simulink library "Surface_Profile_Axle2_KnC"  (R2025a)
settings: Solver=VariableStepAuto  StartTime=0.0  StopTime=10.0  RelTol=1e-3
undefined symbols (not defined in the file): Maneuver
libraries: simulink x2
Description:
  | Simscape Vehicle Templates Library
  | 
  | Copyright 2018-2026 The MathWorks, Inc.
settings Model: Creator=smiller  LastModifiedBy=smiller
settings OptimizationCC: ReuseModelBlockBuffer=off
settings ModelReferenceCC: EnableRefExpFcnMdlSchedulingChecks=on
settings RTWCC: GPUComputeCapability=3.5

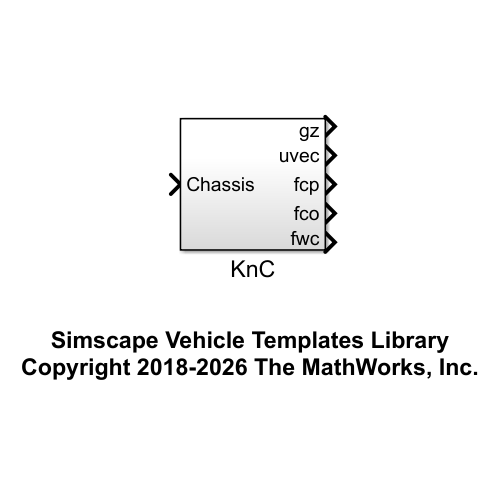
[thumbnail: Simulink's stored preview of the top-level diagram]
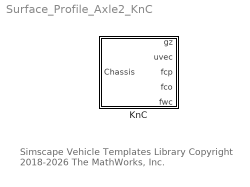
== system Surface_Profile_Axle2_KnC ==
  note: Simscape Vehicle Templates Library
      | Copyright 2018-2026 The MathWorks, Inc.
  KnC : Subsystem  VariantControl=KnC

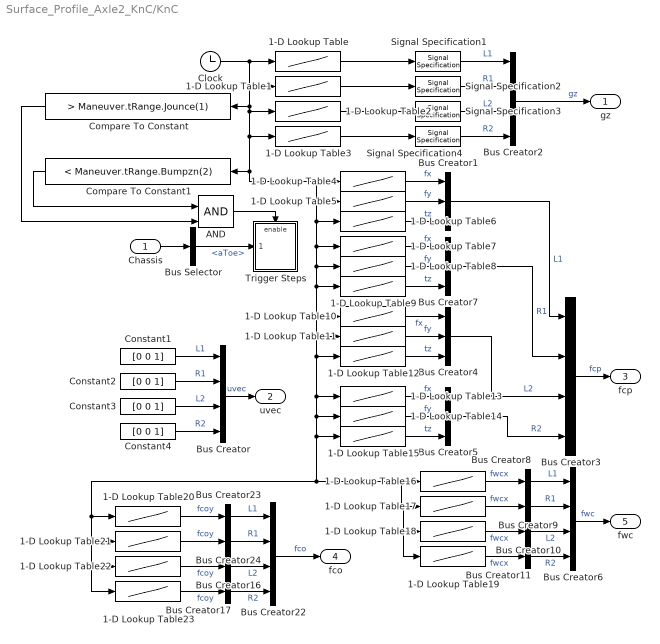
== system Surface_Profile_Axle2_KnC/KnC ==
  Chassis : Inport
  1-D Lookup Table : Lookup_n-D  NumberOfTableDimensions=1  BreakpointsForDimension1=Maneuver.PostL1.t.Value  Table=Maneuver.PostL1.z.Value  InternalRulePriority=Speed  RndMeth=Simplest
  1-D Lookup Table1 : Lookup_n-D  NumberOfTableDimensions=1  BreakpointsForDimension1=Maneuver.PostR1.t.Value  Table=Maneuver.PostR1.z.Value  InternalRulePriority=Speed  RndMeth=Simplest
  1-D Lookup Table10 : Lookup_n-D  NumberOfTableDimensions=1  BreakpointsForDimension1=Maneuver.PostL2.t.Value  Table=Maneuver.PostL2.fx.Value  InternalRulePriority=Speed  RndMeth=Simplest
  1-D Lookup Table11 : Lookup_n-D  NumberOfTableDimensions=1  BreakpointsForDimension1=Maneuver.PostL2.t.Value  Table=Maneuver.PostL2.fy.Value  InternalRulePriority=Speed  RndMeth=Simplest
  1-D Lookup Table12 : Lookup_n-D  NumberOfTableDimensions=1  BreakpointsForDimension1=Maneuver.PostL2.t.Value  Table=Maneuver.PostL2.tz.Value  InternalRulePriority=Speed  RndMeth=Simplest
  1-D Lookup Table13 : Lookup_n-D  NumberOfTableDimensions=1  BreakpointsForDimension1=Maneuver.PostR2.t.Value  Table=Maneuver.PostR2.fx.Value  InternalRulePriority=Speed  RndMeth=Simplest
  1-D Lookup Table14 : Lookup_n-D  NumberOfTableDimensions=1  BreakpointsForDimension1=Maneuver.PostR2.t.Value  Table=Maneuver.PostR2.fy.Value  InternalRulePriority=Speed  RndMeth=Simplest
  1-D Lookup Table15 : Lookup_n-D  NumberOfTableDimensions=1  BreakpointsForDimension1=Maneuver.PostR2.t.Value  Table=Maneuver.PostR2.tz.Value  InternalRulePriority=Speed  RndMeth=Simplest
  1-D Lookup Table16 : Lookup_n-D  NumberOfTableDimensions=1  BreakpointsForDimension1=Maneuver.PostL1.t.Value  Table=Maneuver.PostL1.fwcx.Value  InternalRulePriority=Speed  RndMeth=Simplest
  1-D Lookup Table17 : Lookup_n-D  NumberOfTableDimensions=1  BreakpointsForDimension1=Maneuver.PostR1.t.Value  Table=Maneuver.PostR1.fwcx.Value  InternalRulePriority=Speed  RndMeth=Simplest
  1-D Lookup Table18 : Lookup_n-D  NumberOfTableDimensions=1  BreakpointsForDimension1=Maneuver.PostL2.t.Value  Table=Maneuver.PostL2.fwcx.Value  InternalRulePriority=Speed  RndMeth=Simplest
  1-D Lookup Table19 : Lookup_n-D  NumberOfTableDimensions=1  BreakpointsForDimension1=Maneuver.PostL2.t.Value  Table=Maneuver.PostL2.fwcx.Value  InternalRulePriority=Speed  RndMeth=Simplest
  1-D Lookup Table2 : Lookup_n-D  NumberOfTableDimensions=1  BreakpointsForDimension1=Maneuver.PostL2.t.Value  Table=Maneuver.PostL2.z.Value  InternalRulePriority=Speed  RndMeth=Simplest
  1-D Lookup Table20 : Lookup_n-D  NumberOfTableDimensions=1  BreakpointsForDimension1=Maneuver.PostL1.t.Value  Table=Maneuver.PostL1.fcoy.Value  InternalRulePriority=Speed  RndMeth=Simplest
  1-D Lookup Table21 : Lookup_n-D  NumberOfTableDimensions=1  BreakpointsForDimension1=Maneuver.PostR1.t.Value  Table=Maneuver.PostR1.fcoy.Value  InternalRulePriority=Speed  RndMeth=Simplest
  1-D Lookup Table22 : Lookup_n-D  NumberOfTableDimensions=1  BreakpointsForDimension1=Maneuver.PostL2.t.Value  Table=Maneuver.PostL2.fcoy.Value  InternalRulePriority=Speed  RndMeth=Simplest
  1-D Lookup Table23 : Lookup_n-D  NumberOfTableDimensions=1  BreakpointsForDimension1=Maneuver.PostR2.t.Value  Table=Maneuver.PostR2.fcoy.Value  InternalRulePriority=Speed  RndMeth=Simplest
  1-D Lookup Table3 : Lookup_n-D  NumberOfTableDimensions=1  BreakpointsForDimension1=Maneuver.PostR2.t.Value  Table=Maneuver.PostR2.z.Value  InternalRulePriority=Speed  RndMeth=Simplest
  1-D Lookup Table4 : Lookup_n-D  NumberOfTableDimensions=1  BreakpointsForDimension1=Maneuver.PostL1.t.Value  Table=Maneuver.PostL1.fx.Value  InternalRulePriority=Speed  RndMeth=Simplest
  1-D Lookup Table5 : Lookup_n-D  NumberOfTableDimensions=1  BreakpointsForDimension1=Maneuver.PostL1.t.Value  Table=Maneuver.PostL1.fy.Value  InternalRulePriority=Speed  RndMeth=Simplest
  1-D Lookup Table6 : Lookup_n-D  NumberOfTableDimensions=1  BreakpointsForDimension1=Maneuver.PostL1.t.Value  Table=Maneuver.PostL1.tz.Value  InternalRulePriority=Speed  RndMeth=Simplest
  1-D Lookup Table7 : Lookup_n-D  NumberOfTableDimensions=1  BreakpointsForDimension1=Maneuver.PostR1.t.Value  Table=Maneuver.PostR1.fx.Value  InternalRulePriority=Speed  RndMeth=Simplest
  1-D Lookup Table8 : Lookup_n-D  NumberOfTableDimensions=1  BreakpointsForDimension1=Maneuver.PostR1.t.Value  Table=Maneuver.PostR1.fy.Value  InternalRulePriority=Speed  RndMeth=Simplest
  1-D Lookup Table9 : Lookup_n-D  NumberOfTableDimensions=1  BreakpointsForDimension1=Maneuver.PostR1.t.Value  Table=Maneuver.PostR1.tz.Value  InternalRulePriority=Speed  RndMeth=Simplest
  AND : Logic  IconShape=distinctive  AllPortsSameDT=off  OutDataTypeStr=boolean
  Bus Creator{,2..3,6,22} (5 alike) : BusCreator  Inputs=4
  Bus Creator{1,4..5,7} (4 alike) : BusCreator  Inputs=3
  Bus Creator{8..11,16..17,23..24} (8 alike) : BusCreator  Inputs=1
  Bus Selector : BusSelector  OutputSignals=SuspA1.WhlL.aToe
  Clock : Clock
  Compare To Constant : simulink/Logic and Bit Operations/Compare To Constant  relop=>  const=Maneuver.tRange.Jounce(1)  OutDataTypeStr=boolean  ZeroCross=off
  Compare To Constant1 : simulink/Logic and Bit Operations/Compare To Constant  relop=<  const=Maneuver.tRange.Bumpzn(2)  OutDataTypeStr=boolean  ZeroCross=off
  Constant{1..4} (4 alike) : Constant  Value=[0 0 1]
  Signal Specification{1..4} (4 alike) : SignalSpecification  Unit=m
  Trigger Steps : Subsystem
  gz : Outport  VectorParamsAs1DForOutWhenUnconnected=off
  uvec : Outport  Port=2  VectorParamsAs1DForOutWhenUnconnected=off
  fcp : Outport  Port=3  VectorParamsAs1DForOutWhenUnconnected=off
  fco : Outport  Port=4  VectorParamsAs1DForOutWhenUnconnected=off
  fwc : Outport  Port=5  VectorParamsAs1DForOutWhenUnconnected=off
  wires:
  1-D Lookup Table5/1 -> Bus Creator1/2  "fy"
  1-D Lookup Table4/1 -> Bus Creator1/1  "fx"
  Bus Creator5/1 -> Bus Creator3/4  "R2"
  Bus Creator4/1 -> Bus Creator3/3  "L2"
  Bus Creator1/1 -> Bus Creator3/1  "L1"
  Bus Creator7/1 -> Bus Creator3/2  "R1"
  Bus Creator3/1 -> fcp/1  "fcp"
  1-D Lookup Table3/1 -> Signal Specification4/1
  1-D Lookup Table2/1 -> Signal Specification3/1
  1-D Lookup Table1/1 -> Signal Specification2/1
  1-D Lookup Table/1 -> Signal Specification1/1
  Clock/1 -> 1-D Lookup Table/1, 1-D Lookup Table1/1, Compare To Constant1/1, 1-D Lookup Table23/1, 1-D Lookup Table22/1, 1-D Lookup Table21/1, 1-D Lookup Table20/1, 1-D Lookup Table19/1, 1-D Lookup Table18/1, 1-D Lookup Table17/1, 1-D Lookup Table16/1, 1-D Lookup Table15/1, 1-D Lookup Table14/1, 1-D Lookup Table13/1, 1-D Lookup Table12/1, 1-D Lookup Table11/1, 1-D Lookup Table10/1, 1-D Lookup Table9/1, 1-D Lookup Table8/1, 1-D Lookup Table7/1, 1-D Lookup Table6/1, 1-D Lookup Table5/1, 1-D Lookup Table4/1, 1-D Lookup Table3/1, 1-D Lookup Table2/1, Compare To Constant/1
  Constant4/1 -> Bus Creator/4  "R2"
  Bus Creator/1 -> uvec/1  "uvec"
  Constant1/1 -> Bus Creator/1  "L1"
  Constant2/1 -> Bus Creator/2  "R1"
  Constant3/1 -> Bus Creator/3  "L2"
  Bus Creator2/1 -> gz/1  "gz"
  Signal Specification4/1 -> Bus Creator2/4  "R2"
  Signal Specification1/1 -> Bus Creator2/1  "L1"
  Signal Specification3/1 -> Bus Creator2/3  "L2"
  Signal Specification2/1 -> Bus Creator2/2  "R1"
  Chassis/1 -> Bus Selector/1
  Bus Selector/1 -> Trigger Steps/1(<aToe>)  "<aToe>"
  Compare To Constant/1 -> AND/2
  1-D Lookup Table6/1 -> Bus Creator1/3  "tz"
  1-D Lookup Table7/1 -> Bus Creator7/1  "fx"
  1-D Lookup Table8/1 -> Bus Creator7/2  "fy"
  1-D Lookup Table9/1 -> Bus Creator7/3  "tz"
  1-D Lookup Table12/1 -> Bus Creator4/3  "tz"
  1-D Lookup Table11/1 -> Bus Creator4/2  "fy"
  1-D Lookup Table10/1 -> Bus Creator4/1  "fx"
  1-D Lookup Table13/1 -> Bus Creator5/1  "fx"
  1-D Lookup Table14/1 -> Bus Creator5/2  "fy"
  1-D Lookup Table15/1 -> Bus Creator5/3  "tz"
  Compare To Constant1/1 -> AND/1
  AND/1 -> Trigger Steps/Enable
  Bus Creator6/1 -> fwc/1  "fwc"
  Bus Creator8/1 -> Bus Creator6/1  "L1"
  Bus Creator9/1 -> Bus Creator6/2  "R1"
  Bus Creator10/1 -> Bus Creator6/3  "L2"
  Bus Creator11/1 -> Bus Creator6/4  "R2"
  1-D Lookup Table17/1 -> Bus Creator9/1  "fwcx"
  1-D Lookup Table23/1 -> Bus Creator17/1  "fcoy"
  1-D Lookup Table22/1 -> Bus Creator16/1  "fcoy"
  1-D Lookup Table21/1 -> Bus Creator24/1  "fcoy"
  1-D Lookup Table20/1 -> Bus Creator23/1  "fcoy"
  Bus Creator17/1 -> Bus Creator22/4  "R2"
  Bus Creator16/1 -> Bus Creator22/3  "L2"
  Bus Creator24/1 -> Bus Creator22/2  "R1"
  Bus Creator23/1 -> Bus Creator22/1  "L1"
  Bus Creator22/1 -> fco/1  "fco"
  1-D Lookup Table16/1 -> Bus Creator8/1  "fwcx"
  1-D Lookup Table18/1 -> Bus Creator10/1  "fwcx"
  1-D Lookup Table19/1 -> Bus Creator11/1  "fwcx"

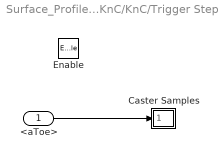
== system Surface_Profile_Axle2_KnC/KnC/Trigger Steps ==
  <aToe> : Inport
  Enable : EnablePort
  Caster Samples : Subsystem  mask{qToe=1}
      mask prompts: qToe "Toe Angle for Caster Measurement (deg)"
  wires:
  <aToe>/1 -> Caster Samples/1(qt)

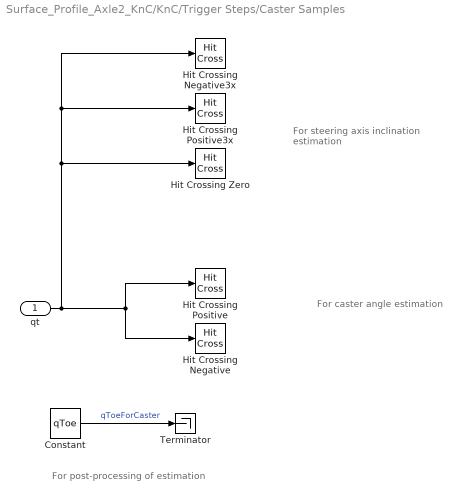
== system Surface_Profile_Axle2_KnC/KnC/Trigger Steps/Caster Samples ==
  note: For post-processing of estimation
  note: For caster angle estimation
  note: For steering axis inclination estimation
  qt : Inport
  Constant : Constant  Value=qToe
  Hit Crossing Negative : HitCross  HitCrossingOffset=-qToe  HitCrossingDirection=falling  ShowOutputPort=off
  Hit Crossing Negative3x : HitCross  HitCrossingOffset=-qToe*3  HitCrossingDirection=falling  ShowOutputPort=off
  Hit Crossing Positive : HitCross  HitCrossingOffset=qToe  HitCrossingDirection=rising  ShowOutputPort=off
  Hit Crossing Positive3x : HitCross  HitCrossingOffset=qToe*3  HitCrossingDirection=rising  ShowOutputPort=off
  Hit Crossing Zero : HitCross  HitCrossingDirection=rising  ShowOutputPort=off
  Terminator : Terminator
  wires:
  qt/1 -> Hit Crossing Positive/1, Hit Crossing Negative/1, Hit Crossing Negative3x/1, Hit Crossing Positive3x/1, Hit Crossing Zero/1
  Constant/1 -> Terminator/1  "qToeForCaster"
